simulink model "three_loop_closed_sim"  (R2023b)
settings: Solver=FixedStepDiscrete  StartTime=0  StopTime=1.2  FixedStep=1e-05  RelTol=1e-3
values from neighbouring files (symbols this model uses):
  A = D{1}    [run_closed_sim.m]
libraries: spsCurrentMeasurementLib x3, spsControlledVoltageSourceLib x3, spsGroundLib x1, spsPermanentMagnetSynchronousMachineLib x1, spspowerguiLib x1
settings Model: Creator=92714  LastModifiedBy=92714
settings DataIOCC: SaveOutput=off  SignalLogging=off

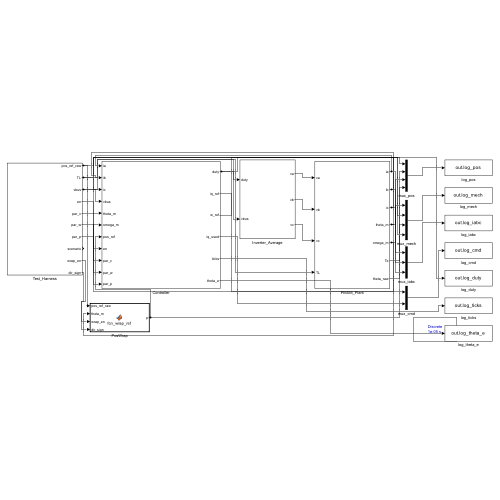
[thumbnail: Simulink's stored preview of the top-level diagram]
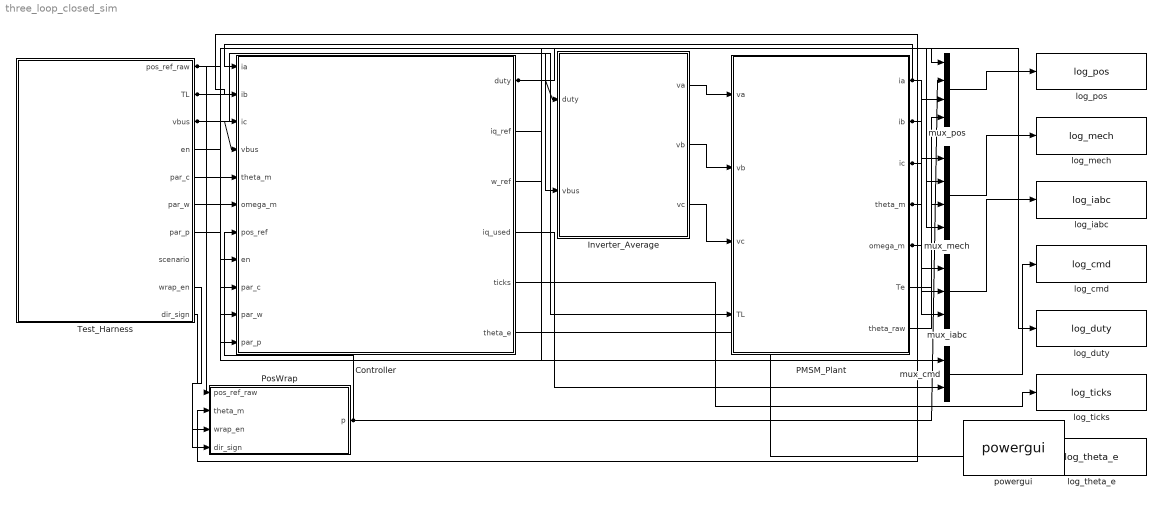
== system three_loop_closed_sim ==
  Controller : Subsystem
  Inverter_Average : Subsystem
  PMSM_Plant : Subsystem
  PosWrap : MATLAB Function  TreatAsAtomicUnit=on  SystemSampleTime=1e-05
  Test_Harness : Subsystem
  log_cmd : ToWorkspace  VariableName=log_cmd  SaveFormat=Timeseries  SampleTime=1e-05
  log_duty : ToWorkspace  VariableName=log_duty  SaveFormat=Timeseries  SampleTime=1e-05
  log_iabc : ToWorkspace  VariableName=log_iabc  SaveFormat=Timeseries  SampleTime=1e-05
  log_mech : ToWorkspace  VariableName=log_mech  SaveFormat=Timeseries  SampleTime=1e-05
  log_pos : ToWorkspace  VariableName=log_pos  SaveFormat=Timeseries  SampleTime=1e-05
  log_theta_e : ToWorkspace  VariableName=log_theta_e  SaveFormat=Timeseries  SampleTime=1e-05
  log_ticks : ToWorkspace  VariableName=log_ticks  SaveFormat=Timeseries  SampleTime=1e-05
  mux_cmd : Mux  Inputs=2
  mux_iabc : Mux  Inputs=3
  mux_mech : Mux
  mux_pos : Mux
  powergui : spspowerguiLib/powergui  Priority=1  SimulationMode=Discrete  SampleTime=1e-05  frequency=60  Iterations=50  frequencyindice=60  Pbase=100e6  ErrMax=1e-4  UnitsV=kV  UnitsW=MW  buscounter=0  FunctionMessages=off  echomessages=off  EnableUseOfTLC=off  CurrentSourceSwitches=off  DisableSnubberDevices=off  DisableRonSwitches=off  DisableVfSwitches=off  DisplayEquations=off  AutomaticDiscreteSolvers=off  SolverType=Tustin/Backward Euler (TBE)  Interpol=off  ExternalGateDelay=off  methode=off  Ts=100  x0status=blocks  SPID=on  SwTol=0  HookPort=off  NonlinearTolerance=1e-4  nMaxIteration=100  ContinueOnMaxIteration=off  RestoreLinks=warning  ResistiveCurrentMeasurement=off  Frange=[0:2:500]  Ylog=off  Xlog=on  ShowGrid=off  save=off  variable=ZData  structure=0  ZoomFFT=off  StartTime=0.0  cycles=1  DisplayStyle=1  fundamental=60  FreqAxis=off  MaxFrequency=1000  frequencyindicesteady=1  RmsSteady=1  display=off
  wires:
  Test_Harness/1(pos_ref_raw) -> PosWrap/1(pos_ref_raw), mux_pos/1
  PMSM_Plant/4(theta_m) -> PosWrap/2(theta_m), Controller/5(theta_m), mux_pos/3
  Test_Harness/9(wrap_en) -> PosWrap/3(wrap_en)
  Test_Harness/10(dir_sign) -> PosWrap/4(dir_sign)
  PosWrap/1(p) -> Controller/7(pos_ref), mux_pos/2
  Test_Harness/2(TL) -> PMSM_Plant/4(TL), mux_mech/4
  Test_Harness/3(vbus) -> Controller/4(vbus), Inverter_Average/2(vbus)
  Test_Harness/4(en) -> Controller/8(en)
  Test_Harness/5(par_c) -> Controller/9(par_c)
  Test_Harness/6(par_w) -> Controller/10(par_w)
  Test_Harness/7(par_p) -> Controller/11(par_p)
  PMSM_Plant/1(ia) -> Controller/1(ia), mux_iabc/1
  PMSM_Plant/2(ib) -> Controller/2(ib), mux_iabc/2
  PMSM_Plant/3(ic) -> Controller/3(ic), mux_iabc/3
  PMSM_Plant/5(omega_m) -> Controller/6(omega_m), mux_mech/1
  Controller/1(duty) -> Inverter_Average/1(duty), log_duty/1
  Inverter_Average/1(va) -> PMSM_Plant/1(va)
  Inverter_Average/2(vb) -> PMSM_Plant/2(vb)
  Inverter_Average/3(vc) -> PMSM_Plant/3(vc)
  PMSM_Plant/7(theta_raw) -> mux_pos/4
  Controller/3(w_ref) -> mux_mech/2
  PMSM_Plant/6(Te) -> mux_mech/3
  Controller/2(iq_ref) -> mux_cmd/1
  Controller/4(iq_used) -> mux_cmd/2
  mux_pos/1 -> log_pos/1
  mux_mech/1 -> log_mech/1
  mux_iabc/1 -> log_iabc/1
  mux_cmd/1 -> log_cmd/1
  Controller/5(ticks) -> log_ticks/1
  Controller/6(theta_e) -> log_theta_e/1

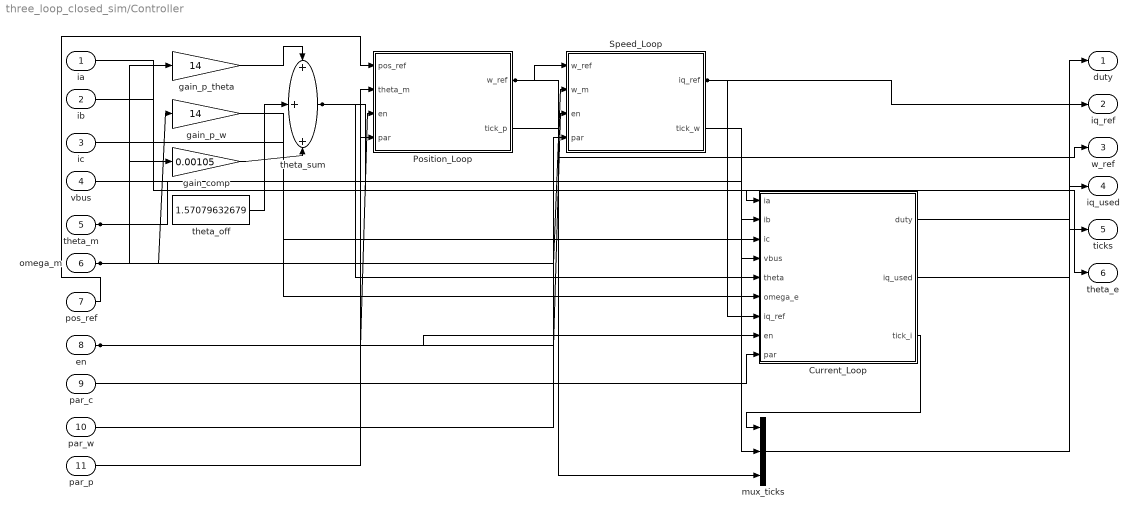
== system three_loop_closed_sim/Controller ==
  ia : Inport
  ib : Inport  Port=2
  ic : Inport  Port=3
  vbus : Inport  Port=4
  theta_m : Inport  Port=5
  omega_m : Inport  Port=6
  pos_ref : Inport  Port=7
  en : Inport  Port=8
  par_c : Inport  Port=9
  par_w : Inport  Port=10
  par_p : Inport  Port=11
  Current_Loop : MATLAB Function  TreatAsAtomicUnit=on  SystemSampleTime=5e-05
  Position_Loop : MATLAB Function  TreatAsAtomicUnit=on  SystemSampleTime=5e-05
  Speed_Loop : MATLAB Function  TreatAsAtomicUnit=on  SystemSampleTime=5e-05
  gain_comp : Gain  Gain=0.00105
  gain_p_theta : Gain  Gain=14
  gain_p_w : Gain  Gain=14
  mux_ticks : Mux  Inputs=3
  theta_off : Constant  Value=1.57079632679
  theta_sum : Sum  Inputs=+++
  duty : Outport
  iq_ref : Outport  Port=2
  w_ref : Outport  Port=3
  iq_used : Outport  Port=4
  ticks : Outport  Port=5
  theta_e : Outport  Port=6
  wires:
  theta_m/1 -> gain_p_theta/1, Position_Loop/2(theta_m)
  omega_m/1 -> gain_p_w/1, gain_comp/1, Speed_Loop/2(w_m)
  gain_p_theta/1 -> theta_sum/1
  theta_off/1 -> theta_sum/2
  gain_comp/1 -> theta_sum/3
  theta_sum/1 -> theta_e/1, Current_Loop/5(theta)
  pos_ref/1 -> Position_Loop/1(pos_ref)
  en/1 -> Position_Loop/3(en), Speed_Loop/3(en), Current_Loop/8(en)
  par_p/1 -> Position_Loop/4(par)
  Position_Loop/1(w_ref) -> w_ref/1, Speed_Loop/1(w_ref)
  Position_Loop/2(tick_p) -> mux_ticks/3
  par_w/1 -> Speed_Loop/4(par)
  Speed_Loop/1(iq_ref) -> iq_ref/1, Current_Loop/7(iq_ref)
  Speed_Loop/2(tick_w) -> mux_ticks/2
  ia/1 -> Current_Loop/1(ia)
  ib/1 -> Current_Loop/2(ib)
  ic/1 -> Current_Loop/3(ic)
  vbus/1 -> Current_Loop/4(vbus)
  gain_p_w/1 -> Current_Loop/6(omega_e)
  par_c/1 -> Current_Loop/9(par)
  Current_Loop/1(duty) -> duty/1
  Current_Loop/2(iq_used) -> iq_used/1
  Current_Loop/3(tick_i) -> mux_ticks/1
  mux_ticks/1 -> ticks/1

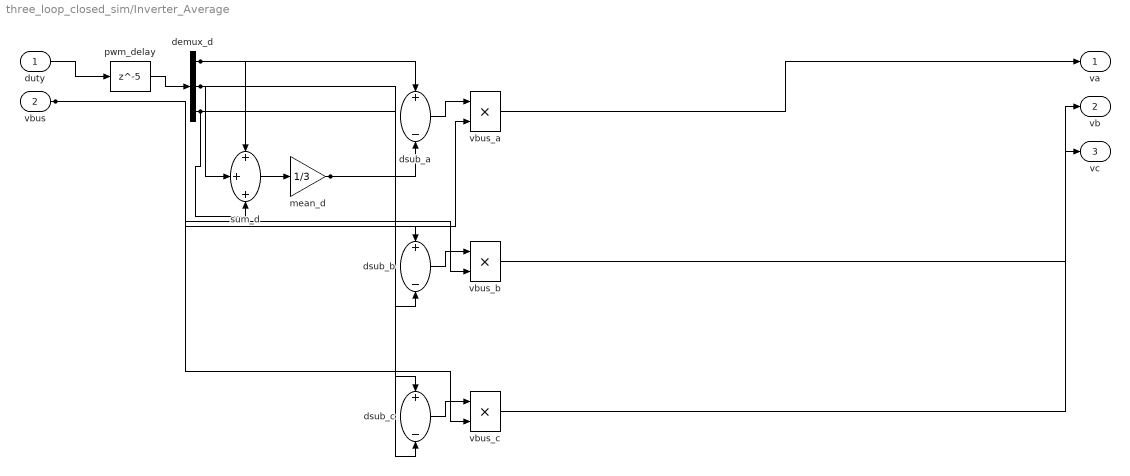
== system three_loop_closed_sim/Inverter_Average ==
  duty : Inport
  vbus : Inport  Port=2
  demux_d : Demux  Outputs=3
  dsub_a : Sum  Inputs=+-
  dsub_b : Sum  Inputs=+-
  dsub_c : Sum  Inputs=+-
  mean_d : Gain  Gain=1/3
  pwm_delay : Delay  DelayLength=5  SampleTime=1e-05
  sum_d : Sum  Inputs=+++
  vbus_a : Product
  vbus_b : Product
  vbus_c : Product
  va : Outport
  vb : Outport  Port=2
  vc : Outport  Port=3
  wires:
  duty/1 -> pwm_delay/1
  pwm_delay/1 -> demux_d/1
  demux_d/1 -> sum_d/1, dsub_a/1
  demux_d/2 -> sum_d/2, dsub_b/1
  demux_d/3 -> sum_d/3, dsub_c/1
  sum_d/1 -> mean_d/1
  mean_d/1 -> dsub_a/2, dsub_b/2, dsub_c/2
  dsub_a/1 -> vbus_a/1
  vbus/1 -> vbus_a/2, vbus_b/2, vbus_c/2
  vbus_a/1 -> va/1
  dsub_b/1 -> vbus_b/1
  vbus_b/1 -> vb/1
  dsub_c/1 -> vbus_c/1
  vbus_c/1 -> vc/1

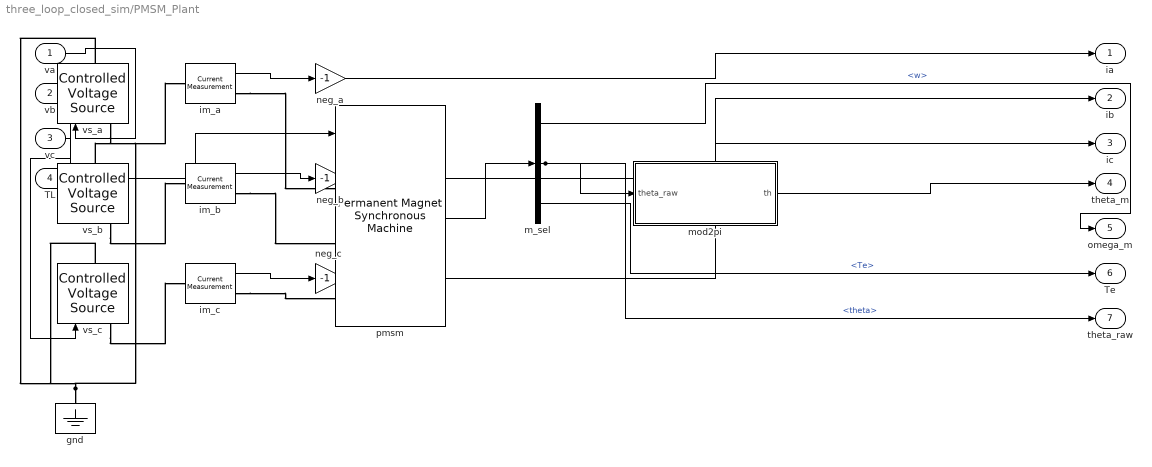
== system three_loop_closed_sim/PMSM_Plant ==
  va : Inport
  vb : Inport  Port=2
  vc : Inport  Port=3
  TL : Inport  Port=4
  gnd : spsGroundLib/Ground  LConnTagsString=a
  im_a : spsCurrentMeasurementLib/Current Measurement  PhasorSimulation=off  OutputType=Complex  PSBequivalent=0
  im_b : spsCurrentMeasurementLib/Current Measurement  PhasorSimulation=off  OutputType=Complex  PSBequivalent=0
  im_c : spsCurrentMeasurementLib/Current Measurement  PhasorSimulation=off  OutputType=Complex  PSBequivalent=0
  m_sel : BusSelector  OutputSignals=w,theta,Te
  mod2pi : MATLAB Function  TreatAsAtomicUnit=on  SystemSampleTime=1e-05
  neg_a : Gain  Gain=-1
  neg_b : Gain  Gain=-1
  neg_c : Gain  Gain=-1
  pmsm : spsPermanentMagnetSynchronousMachineLib/Permanent Magnet Synchronous Machine  NbPhases=3  FluxDistribution=Sinusoidal  RotorType=Round  MechanicalLoad=Torque Tm  PresetModel=No  ShowDetailedParameters=on  MeasurementBus=on  Resistance=0.3785  Inductance=8.5e-3  dqInductances=[0.0001135 0.0001135]  La=0.000395  MachineConstant=Flux linkage established by magnets (V.s)  Flux=0.00759297995988  VoltageCst=19.281  TorqueCst=0.15945  Flat=120  Mechanical=[2.5725e-05 1e-05 14 0]  PolePairs=4  InitialConditions=[0,0, 0,0]  InitialConditions5ph=[0 0 0 0 0 0]  RefAngle=90 degrees behind phase A axis (modified Park)  IterativeDiscreteModel=Trapezoidal non iterative  TsBlock=-1  TsPowergui=0
  vs_a : spsControlledVoltageSourceLib/Controlled Voltage Source  Initialize=on  Source_Type=AC  Amplitude=0  Phase=0  Frequency=0  Measurements=None
  vs_b : spsControlledVoltageSourceLib/Controlled Voltage Source  Initialize=on  Source_Type=AC  Amplitude=0  Phase=0  Frequency=0  Measurements=None
  vs_c : spsControlledVoltageSourceLib/Controlled Voltage Source  Initialize=on  Source_Type=AC  Amplitude=0  Phase=0  Frequency=0  Measurements=None
  ia : Outport
  ib : Outport  Port=2
  ic : Outport  Port=3
  theta_m : Outport  Port=4
  omega_m : Outport  Port=5
  Te : Outport  Port=6
  theta_raw : Outport  Port=7
  wires:
  va/1 -> vs_a/1
  vb/1 -> vs_b/1
  vc/1 -> vs_c/1
  TL/1 -> pmsm/1
  pmsm/1 -> m_sel/1
  im_a/1 -> neg_a/1
  im_b/1 -> neg_b/1
  im_c/1 -> neg_c/1
  neg_a/1 -> ia/1
  neg_b/1 -> ib/1
  neg_c/1 -> ic/1
  m_sel/1 -> omega_m/1  "<w>"
  m_sel/2 -> theta_raw/1, mod2pi/1(theta_raw)  "<theta>"
  mod2pi/1(th) -> theta_m/1
  m_sel/3 -> Te/1  "<Te>"
  connections:
  vs_a/LConn1 -- im_a/LConn1
  vs_b/LConn1 -- im_b/LConn1
  vs_c/LConn1 -- im_c/LConn1
  im_a/RConn1 -- pmsm/LConn1
  im_b/RConn1 -- pmsm/LConn2
  im_c/RConn1 -- pmsm/LConn3
  vs_a/RConn1 -- vs_b/RConn1 -- gnd/LConn1 -- vs_c/RConn1

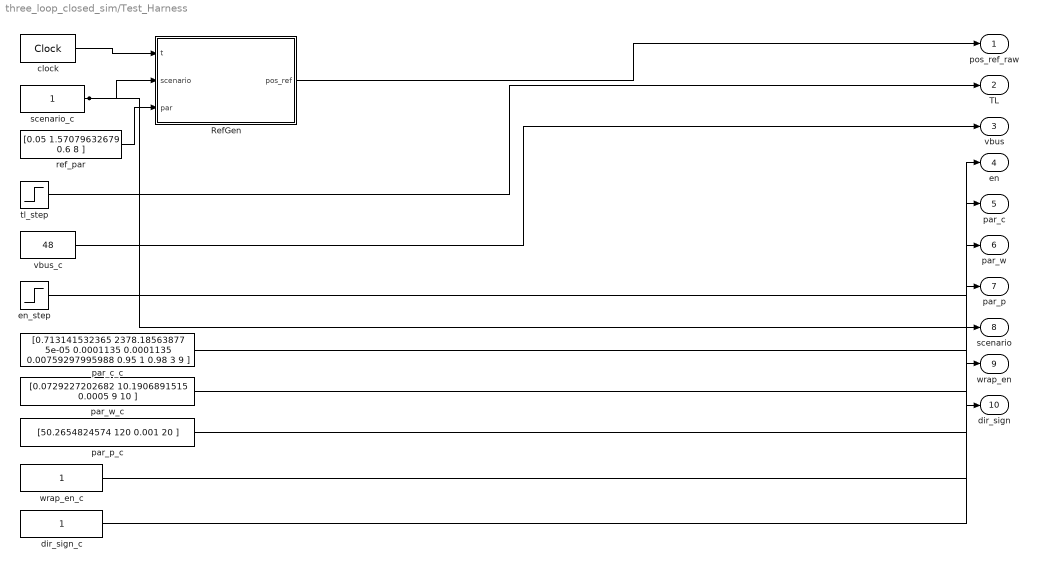
== system three_loop_closed_sim/Test_Harness ==
  RefGen : MATLAB Function  TreatAsAtomicUnit=on  SystemSampleTime=1e-05
  clock : DigitalClock  SampleTime=1e-05
  dir_sign_c : Constant
  en_step : Step  Time=0.005  SampleTime=5e-05
  par_c_c : Constant  Value=[0.713141532365 2378.18563877 5e-05 0.0001135 0.0001135 0.00759297995988 0.95 1 0.98 3 9 ]
  par_p_c : Constant  Value=[50.2654824574 120 0.001 20 ]
  par_w_c : Constant  Value=[0.0729227202682 10.1906891515 0.0005 9 10 ]
  ref_par : Constant  Value=[0.05 1.57079632679 0.6 8 ]
  scenario_c : Constant
  tl_step : Step  Time=0.35  After=0.05  SampleTime=1e-05
  vbus_c : Constant  Value=48
  wrap_en_c : Constant
  pos_ref_raw : Outport
  TL : Outport  Port=2
  vbus : Outport  Port=3
  en : Outport  Port=4
  par_c : Outport  Port=5
  par_w : Outport  Port=6
  par_p : Outport  Port=7
  scenario : Outport  Port=8
  wrap_en : Outport  Port=9
  dir_sign : Outport  Port=10
  wires:
  clock/1 -> RefGen/1(t)
  scenario_c/1 -> RefGen/2(scenario), scenario/1
  ref_par/1 -> RefGen/3(par)
  RefGen/1(pos_ref) -> pos_ref_raw/1
  tl_step/1 -> TL/1
  vbus_c/1 -> vbus/1
  en_step/1 -> en/1
  par_c_c/1 -> par_c/1
  par_w_c/1 -> par_w/1
  par_p_c/1 -> par_p/1
  wrap_en_c/1 -> wrap_en/1
  dir_sign_c/1 -> dir_sign/1

== matlab function three_loop_closed_sim/Controller/Position_Loop ==
  data: pos_ref input; w_ref output; theta_m input; en input; par input; tick_p output
function [w_ref, tick_p] = fcn_three_pos_loop_deploy(pos_ref, theta_m, en, par)
%FCN_THREE_POS_LOOP_DEPLOY  位置环 P（部署版，单 50us ISR 内部分频到 1 kHz）
%
% MCU 部署模型运行在单一 20 kHz 节拍上；本函数每 N_div=20 拍真正计算一次，
% 其余拍保持上次输出（ZOH），因此等效执行频率 = 20 kHz / 20 = 1 kHz。
%
% par = [kp_p, w_max, Ts_p, N_div_p]
%   kp_p    [(rad/s)/rad]  = 50.265482
%   w_max   [rad/s]        位置环输出限速
%   Ts_p    [s]            1 ms（仅用于文档/核对，P 环不用 dt）
%   N_div_p 分频系数        = Ts_p/Ts_i = 20
%
% tick_p：实际执行次数（每计算一次 +1），用于在线核对 1 kHz 执行频率。

%#codegen
persistent cnt hold_w n_exec
if isempty(cnt)
    cnt    = 0.0;
    hold_w = 0.0;
    n_exec = 0.0;
end

kp    = par(1);
w_max = par(2);
n_div = par(4);

if en < 0.5
    % 关断立即清零输出，不等分频点（安全要求）
    hold_w = 0.0;
else
    cnt = cnt + 1.0;
    if cnt >= n_div
        cnt    = 0.0;
        n_exec = n_exec + 1.0;
        w = kp * (pos_ref - theta_m);
        if w > w_max
            w = w_max;
        elseif w < -w_max
            w = -w_max;
        end
        hold_w = w;
    end
end

w_ref  = hold_w;
tick_p = n_exec;
end

== matlab function three_loop_closed_sim/Test_Harness/RefGen ==
  data: t input; pos_ref output; scenario input; par input
function pos_ref = fcn_ref_gen(t, scenario, par)
%FCN_REF_GEN  位置指令发生器
%  scenario = 1: 位置阶跃 0 -> +90deg @0.05s，0.60s 回零
%  scenario = 2: 连续旋转多圈累积指令 pos_ref = vel_ref * t（速度模式，用于跨 2pi 验证）
%  par = [pos_t1, pos_a1, pos_t2, vel_ref]

%#codegen
pos_ref = 0.0;

if scenario < 1.5
    if t >= par(1)
        pos_ref = pos_ref + par(2);
    end
    if t >= par(3)
        pos_ref = pos_ref - par(2);
    end
else
    pos_ref = par(4) * t;
end
end

== matlab function three_loop_closed_sim/Controller/Speed_Loop ==
  data: w_ref input; iq_ref output; w_m input; en input; par input; tick_w output
function [iq_ref, tick_w] = fcn_three_speed_loop_deploy(w_ref, w_m, en, par)
%FCN_THREE_SPEED_LOOP_DEPLOY  速度环 PI（部署版，单 50us ISR 内部分频到 2 kHz）
%
% 每 N_div=10 拍真正计算一次（等效 2 kHz），其余拍保持输出。
% PI 积分步长用 Ts_w = 500 us，与仿真模型的 2 kHz 速度环完全一致。
%
% par = [kp_w, ki_w, Ts_w, i_max, N_div_w]
%   kp_w [A/(rad/s)] = 0.072923
%   ki_w [A/(rad/s)/s] = 10.190689
%   Ts_w = 500 us
%   i_max = 9 A
%   N_div_w = Ts_w/Ts_i = 10
%
% tick_w：实际执行次数，用于在线核对 2 kHz 执行频率。

%#codegen
persistent i_term cnt hold_iq n_exec
if isempty(i_term)
    i_term   = 0.0;
    cnt      = 0.0;
    hold_iq  = 0.0;
    n_exec   = 0.0;
end

kp    = par(1);
ki    = par(2);
ts    = par(3);
i_max = par(4);
n_div = par(5);

if en < 0.5
    i_term  = 0.0;
    hold_iq = 0.0;
else
    cnt = cnt + 1.0;
    if cnt >= n_div
        cnt    = 0.0;
        n_exec = n_exec + 1.0;

        err = w_ref - w_m;
        i_term = i_term + ki * err * ts;
        if i_term > i_max
            i_term = i_max;
        elseif i_term < -i_max
            i_term = -i_max;
        end

        out = kp * err + i_term;
        if out > i_max
            out = i_max;
        elseif out < -i_max
            out = -i_max;
        end
        hold_iq = out;
    end
end

iq_ref = hold_iq;
tick_w = n_exec;
end

== matlab function three_loop_closed_sim/Controller/Current_Loop ==
  data: ia input; duty output; ib input; ic input; vbus input; theta input; omega_e input; iq_ref input; en input; par input; iq_used output; tick_i output
function [duty, iq_used, tick_i] = fcn_three_current_loop_deploy(ia, ib, ic, vbus, theta, omega_e, iq_ref, en, par)
%FCN_THREE_CURRENT_LOOP_DEPLOY  有感 FOC 电流环（部署版，20 kHz 每拍执行）
%
% 与仿真模型 three_loop_pmsm_sim 的电流环逐行一致：
%   Clarke(幅值不变) -> Park -> dq PI(积分先行) -> 交叉耦合/BEMF 全解耦
%   -> 电压圆限幅(d 优先) -> 归一化 -> 反 Park -> SVPWM 六扇区 -> 三相占空比
%
% par = [kp ki dt Ld Lq psi max_duty overmod mag_vd_max dec imax]
%   kp=0.713142 V/A, ki=2378.186 V/(A*s), dt=50us, Ld=Lq=113.5uH,
%   psi=7.593mWb, max_duty=0.95, overmod=1, mag_vd_max=0.98, dec=3, imax=9A
%
% 输出 duty 为 3x1 向量 [da db dc] ∈ [0,1]，可直接映射到 TIM1 CCR。
% deploy 版不输出 diagv 向量（避免 ERT 类型推导问题），仅保留 iq_used/tick_i。

%#codegen
persistent vd_int vq_int n_exec
if isempty(vd_int)
    vd_int = 0.0;
    vq_int = 0.0;
    n_exec = 0.0;
end
n_exec = n_exec + 1.0;
tick_i = n_exec;

kp         = par(1);
ki         = par(2);
dt         = par(3);
Ld         = par(4);
Lq         = par(5);
psi        = par(6);
max_duty   = par(7);
overmod    = par(8);
mag_vd_max = par(9);
dec_mode   = par(10);
i_max      = par(11);

ONE_BY_SQRT3 = 0.5773502691896258;
TWO_BY_SQRT3 = 1.1547005383792515;

% ---- Clarke（幅值不变）----
i_alpha = ia;
i_beta  = ONE_BY_SQRT3 * ia + TWO_BY_SQRT3 * ib;

s = sin(theta);
c = cos(theta);

% ---- Park（标准）----
id = c * i_alpha + s * i_beta;
iq = c * i_beta  - s * i_alpha;

% ---- 电流给定限幅 ----
iq_cmd = iq_ref;
if iq_cmd > i_max
    iq_cmd = i_max;
elseif iq_cmd < -i_max
    iq_cmd = -i_max;
end
iq_used = iq_cmd;

vd        = 0.0;
vq        = 0.0;
mod_alpha = 0.0;
mod_beta  = 0.0;
sector    = 0.0;
duty      = [0.5; 0.5; 0.5];

if en < 0.5
    vd_int = 0.0;
    vq_int = 0.0;
else
    err_d = 0.0 - id;
    err_q = iq_cmd - iq;

    % 积分先行，再比例
    vd_int = vd_int + err_d * ki * dt;
    vq_int = vq_int + err_q * ki * dt;

    vd = vd_int + err_d * kp;
    vq = vq_int + err_q * kp;

    % ---- 解耦前馈（dec=3：交叉耦合 + BEMF）----
    dec_vd   = 0.0;
    dec_vq   = 0.0;
    dec_bemf = 0.0;
    if dec_mode == 1 || dec_mode == 3
        dec_vd = iq * omega_e * Lq;
        dec_vq = id * omega_e * Ld;
    end
    if dec_mode == 2 || dec_mode == 3
        dec_bemf = omega_e * psi;
    end
    vd = vd - dec_vd;
    vq = vq + dec_vq + dec_bemf;

    % ---- 电压圆限幅（d 轴优先，积分器同步钳位）----
    max_v_mag = ONE_BY_SQRT3 * max_duty * vbus * overmod;
    lim_d = max_v_mag * mag_vd_max;

    if vd > lim_d
        vd = lim_d;
    elseif vd < -lim_d
        vd = -lim_d;
    end
    if vd_int > lim_d
        vd_int = lim_d;
    elseif vd_int < -lim_d
        vd_int = -lim_d;
    end

    tmp = max_v_mag * max_v_mag - vd * vd;
    if tmp > 0.0
        max_vq = sqrt(tmp);
    else
        max_vq = 0.0;
    end
    if vq > max_vq
        vq = max_vq;
    elseif vq < -max_vq
        vq = -max_vq;
    end
    if vq_int > max_vq
        vq_int = max_vq;
    elseif vq_int < -max_vq
        vq_int = -max_vq;
    end

    % ---- 归一化：mod = v * 1.5 / vbus ----
    vn    = 1.5 / vbus;
    mod_d = vd * vn;
    mod_q = vq * vn;

    % ---- 反 Park（标准）----
    mod_alpha = c * mod_d - s * mod_q;
    mod_beta  = c * mod_q + s * mod_d;

    [duty, sector] = three_svm_deploy(mod_alpha, mod_beta, max_duty);
end
end

% =======================================================================
function [duty, sector] = three_svm_deploy(alpha, beta, max_mod)
%THREE_SVM_DEPLOY  SVPWM 六扇区 + 归一化占空比

ONE_BY_SQRT3 = 0.5773502691896258;
TWO_BY_SQRT3 = 1.1547005383792515;

if beta >= 0.0
    if alpha >= 0.0
        if ONE_BY_SQRT3 * beta > alpha
            sector = 2;
        else
            sector = 1;
        end
    else
        if -ONE_BY_SQRT3 * beta > alpha
            sector = 3;
        else
            sector = 2;
        end
    end
else
    if alpha >= 0.0
        if -ONE_BY_SQRT3 * beta > alpha
            sector = 5;
        else
            sector = 6;
        end
    else
        if ONE_BY_SQRT3 * beta > alpha
            sector = 4;
        else
            sector = 5;
        end
    end
end

dA = 0.5;
dB = 0.5;
dC = 0.5;

if sector == 1
    t1 = alpha - ONE_BY_SQRT3 * beta;
    t2 = TWO_BY_SQRT3 * beta;
    dA = (1.0 + t1 + t2) * 0.5;
    dB = dA - t1;
    dC = dB - t2;
elseif sector == 2
    t2 = alpha + ONE_BY_SQRT3 * beta;
    t3 = -alpha + ONE_BY_SQRT3 * beta;
    dB = (1.0 + t2 + t3) * 0.5;
    dA = dB - t3;
    dC = dA - t2;
elseif sector == 3
    t3 = TWO_BY_SQRT3 * beta;
    t4 = -alpha - ONE_BY_SQRT3 * beta;
    dB = (1.0 + t3 + t4) * 0.5;
    dC = dB - t3;
    dA = dC - t4;
elseif sector == 4
    t4 = -alpha + ONE_BY_SQRT3 * beta;
    t5 = -TWO_BY_SQRT3 * beta;
    dC = (1.0 + t4 + t5) * 0.5;
    dB = dC - t5;
    dA = dB - t4;
elseif sector == 5
    t5 = -alpha - ONE_BY_SQRT3 * beta;
    t6 = alpha - ONE_BY_SQRT3 * beta;
    dC = (1.0 + t5 + t6) * 0.5;
    dA = dC - t5;
    dB = dA - t6;
else
    t6 = -TWO_BY_SQRT3 * beta;
    t1 = alpha + ONE_BY_SQRT3 * beta;
    dA = (1.0 + t1 + t6) * 0.5;
    dC = dA - t1;
    dB = dC - t6;
end

d_max = (1.0 + max_mod) * 0.5;
if dA > d_max
    dA = d_max;
elseif dA < 0.0
    dA = 0.0;
end
if dB > d_max
    dB = d_max;
elseif dB < 0.0
    dB = 0.0;
end
if dC > d_max
    dC = d_max;
elseif dC < 0.0
    dC = 0.0;
end

duty = [dA; dB; dC];
end

== matlab function three_loop_closed_sim/PMSM_Plant/mod2pi ==
  data: theta_raw input; th output
function th = fcn_mod2pi(theta_raw)
%FCN_MOD2PI  把 SPS PMSM 连续累积的机械角折成单圈 0..2pi，
% 模拟真实 MT6835 21bit 绝对编码器（BSP 层会把 theta 折到单圈）。
% p=14 为整数，14*theta 在跳变点相差 28pi = 14*2pi，电角连续，不影响 Park。

%#codegen
TWO_PI = 6.28318530717958647692;
th = mod(theta_raw, TWO_PI);
end

== matlab function three_loop_closed_sim/PosWrap ==
  data: pos_ref_raw input; p output; theta_m input; wrap_en input; dir_sign input
function p = fcn_wrap_ref(pos_ref_raw, theta_m, wrap_en, dir_sign)
%FCN_WRAP_REF  位置指令坐标系折叠（与 three_loop_tuning.c 的 WrapPosRefEx 一致）
%  wrap_en = 0 时不折叠（复现文档 §3.3 的跨 2pi 过流 bug）
%  wrap_en = 1 时把多圈 pos_ref 折到 theta_m 所在圈，误差 = wrap_pi(真实误差)

%#codegen
TWO_PI = 6.28318530717958647692;

if wrap_en < 0.5
    p = pos_ref_raw;
else
    ds = dir_sign;
    if ds >= 0.0
        ds = 1.0;
    else
        ds = -1.0;
    end
    th = ds * theta_m;
    e  = ds * (pos_ref_raw - theta_m);
    e  = e - TWO_PI * floor(e * (1.0/TWO_PI) + 0.5);
    p  = th + e;
end
end
